simulink model "panda_circle_warm"  (R2024b)
settings: Solver=FixedStepDiscrete  StartTime=0.0  StopTime=4  FixedStep=0.02  RelTol=1e-3
values from neighbouring files (symbols this model uses):
  circlePeriod = 4    [task6_init.m]
  circleRadius = 0.10    (= 0.1)    [task6_init.m]
  Tready = getTransform(panda,qReady,ee)    [task5_panda_trajectory.m]    (also in task6_init.m)
  Ts = 0.02    [task6_init.m]
undefined symbols (not defined in the file or in its folder): Levenberg, Marquardt, qCircle0
libraries: robotmaniplib x2
settings Model: Creator=Omen Gaming 16  LastModifiedBy=Omen Gaming 16

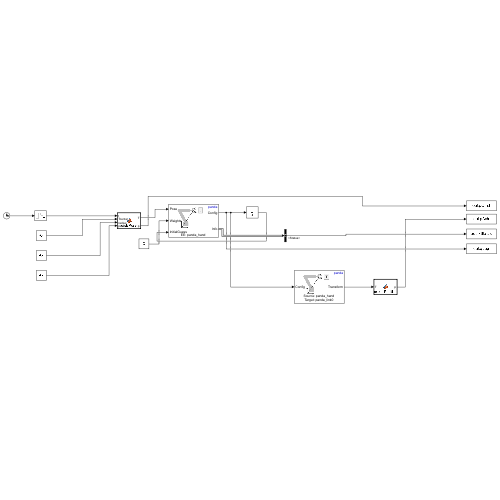
[thumbnail: Simulink's stored preview of the top-level diagram]
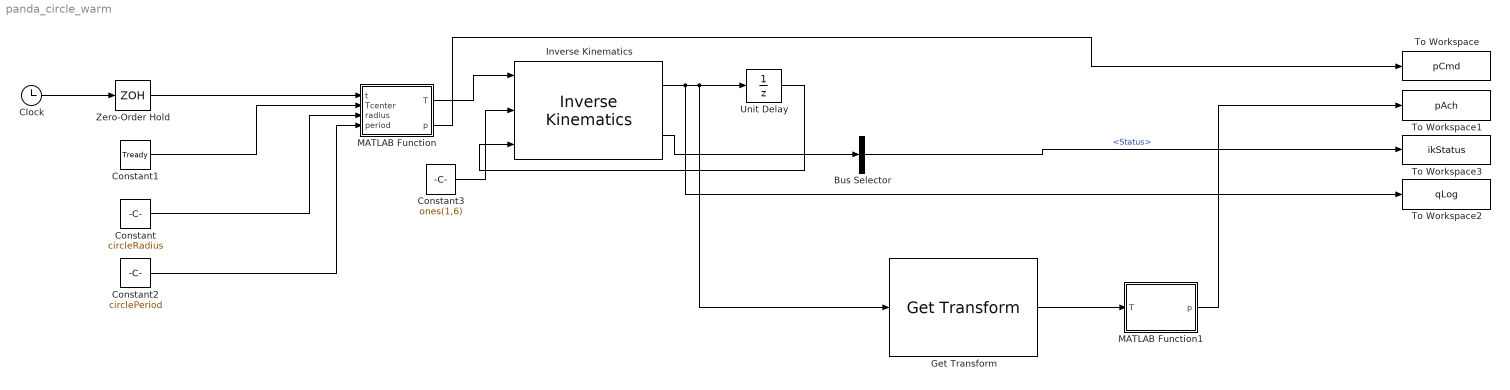
== system panda_circle_warm ==
  Bus Selector : BusSelector  OutputSignals=Status
  Clock : Clock
  Constant : Constant  Value=circleRadius
  Constant1 : Constant  Value=Tready
  Constant2 : Constant  Value=circlePeriod
  Constant3 : Constant  Value=ones(1,6)
  Get Transform : robotmaniplib/Get Transform  RigidBodyTree=panda  SourceBody=panda_hand  TargetBody=panda_link0  SimulateUsing=Interpreted execution
  Inverse Kinematics : robotmaniplib/Inverse Kinematics  RigidBodyTree=panda  EndEffector=panda_hand  ShowInfo=on  SolverName=Levenberg-Marquardt  EnforceJointLimits=on  MaxIterations=500  MaxTime=10  GradientTolerance=1e-12  SolutionTolerance=1e-12  StepTolerance=1e-14  ErrorChangeTolerance=1e-12  UseErrorDamping=on  DampingBias=0.0025  SimulateUsing=Interpreted execution
  MATLAB Function : MATLAB Function  TreatAsAtomicUnit=on
  MATLAB Function1 : MATLAB Function  TreatAsAtomicUnit=on
  To Workspace : ToWorkspace  VariableName=pCmd  SaveFormat=Timeseries  SampleTime=-1
  To Workspace1 : ToWorkspace  VariableName=pAch  SaveFormat=Timeseries  SampleTime=-1
  To Workspace2 : ToWorkspace  VariableName=qLog  SaveFormat=Timeseries  SampleTime=-1
  To Workspace3 : ToWorkspace  VariableName=ikStatus  SaveFormat=Timeseries  SampleTime=-1
  Unit Delay : UnitDelay  InitialCondition=qCircle0  SampleTime=Ts  HasFrameUpgradeWarning=on
  Zero-Order Hold : ZeroOrderHold  SampleTime=Ts
  wires:
  Clock/1 -> Zero-Order Hold/1
  Zero-Order Hold/1 -> MATLAB Function/1(t)
  Constant1/1 -> MATLAB Function/2(Tcenter)
  Constant/1 -> MATLAB Function/3(radius)
  Constant2/1 -> MATLAB Function/4(period)
  MATLAB Function/1(T) -> Inverse Kinematics/1
  Constant3/1 -> Inverse Kinematics/2
  Inverse Kinematics/1 -> To Workspace2/1, Get Transform/1, Unit Delay/1
  Get Transform/1 -> MATLAB Function1/1(T)
  Inverse Kinematics/2 -> Bus Selector/1
  MATLAB Function1/1(p) -> To Workspace1/1
  MATLAB Function/2(p) -> To Workspace/1
  Bus Selector/1 -> To Workspace3/1  "<Status>"
  Unit Delay/1 -> Inverse Kinematics/3

== matlab function panda_circle_warm/MATLAB Function1 ==
  data: T input; p output
function p = extractPosition(T)
% I extract the hand position from its transformation.
p = T(1:3,4);
end

== matlab function panda_circle_warm/MATLAB Function ==
  data: t input; T output; Tcenter input; radius input; period input; p output
function [T,p] = circlePose(t,Tcenter,radius,period)
% I generate a circle while keeping the hand orientation fixed.

angle = 2*pi*t/period;

p = Tcenter(1:3,4) + ...
    [radius*cos(angle);
     radius*sin(angle);
     0];

T = Tcenter;
T(1:3,4) = p;
end
